simulink model "UAV_Load_Balancing_Main"  (R2025b)
settings: Solver=ode23t  StartTime=0.0  StopTime=8  FixedStep=1e-5  MaxStep=1e-5  RelTol=1e-3
libraries: nesl_utility x67, fl_lib x49, ee_lib x36
(part 1 of 2)
settings Model: Creator=cevo_  LastModifiedBy=cevo_

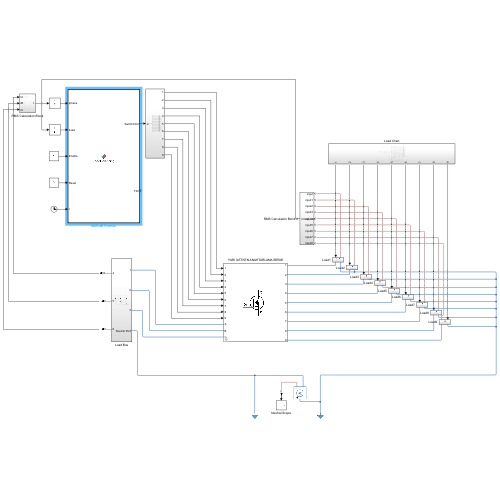
[thumbnail: Simulink's stored preview of the top-level diagram]
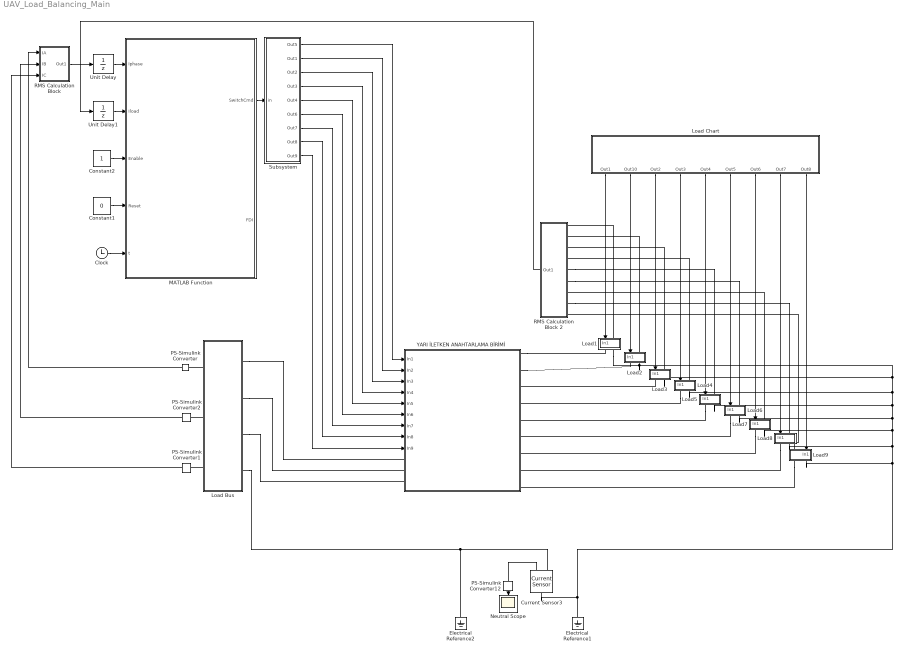
== system UAV_Load_Balancing_Main ==
  Clock : Clock
  Constant1 : Constant  Value=0
  Constant2 : Constant
  Current Sensor3 : fl_lib/Electrical/Electrical Sensors/Current Sensor
  Electrical Reference1 : fl_lib/Electrical/Electrical Elements/Electrical Reference
  Electrical Reference2 : fl_lib/Electrical/Electrical Elements/Electrical Reference
  Load Bus : Subsystem
  Load Chart : Subsystem
  Load1 : Subsystem
  Load2 : Subsystem
  Load3 : Subsystem
  Load4 : Subsystem
  Load5 : Subsystem
  Load6 : Subsystem
  Load7 : Subsystem
  Load8 : Subsystem
  Load9 : Subsystem
      settings: PortSchema="{\"entries\":[{\"content\":{\"sides\":[{\"content\":{\"connectorIds\":[\"LConn1\",\"In1\"]},\"type\":\"ConnectorPlacement.EquallySpacedRectSide\",\"uuid\":\"d3e55c95-e0b0-4c19-a363-030e817358eb\"},{\"content\":{\"connectorIds\":[\"RConn1\",\"RConn2\"],\"side\":\"RIGHT\"},\"type\":\"ConnectorPlacement.EquallySpacedRectSide\",\"uuid\":\"a0e4c3e1-714c-47ca-a01a-393fa4d5956a\"},{\"content\":{\"side\":\"TOP\"},\"type\":\"ConnectorPlacement.EquallySpacedRectSide\",\"uuid\":\"b8c3a6c7-6915-4d93-933f-da8484f2cfda\"}]},\"type\":\"ConnectorPlacement.EquallySpacedConnector\",\"uuid\":\"988140d9-c12a-4da7-b803-ba7ebfbbead4\"}],\"packageUris\":[\"http://schema.mathworks.com/mf0/Connector/R2020b\"],\"version\":\"1.0\"}"
  MATLAB Function : MATLAB Function  TreatAsAtomicUnit=on
  Neutral Scope : Scope
      settings: ActiveDisplayYMinimum=-0.021583988846100941  ActiveDisplayYMaximum=0.036156729353894947  DataLoggingVariableName=ScopeData14
  PS-Simulink Converter : nesl_utility/PS-Simulink Converter  PhysicalDomain=network_engine_domain  SubClassName=ps_output  LeftPortType=input  RightPortType=output  PseudoPeriodic=off  Frequencies=[]  VectorFormat=inherit  Unit=inherit  AffineConversion=off
  PS-Simulink Converter1 : nesl_utility/PS-Simulink Converter  PhysicalDomain=network_engine_domain  SubClassName=ps_output  LeftPortType=input  RightPortType=output  PseudoPeriodic=off  Frequencies=[]  VectorFormat=inherit  Unit=inherit  AffineConversion=off
  PS-Simulink Converter12 : nesl_utility/PS-Simulink Converter  PhysicalDomain=network_engine_domain  SubClassName=ps_output  LeftPortType=input  RightPortType=output  PseudoPeriodic=off  Frequencies=[]  VectorFormat=inherit  Unit=A  AffineConversion=off
  PS-Simulink Converter2 : nesl_utility/PS-Simulink Converter  PhysicalDomain=network_engine_domain  SubClassName=ps_output  LeftPortType=input  RightPortType=output  PseudoPeriodic=off  Frequencies=[]  VectorFormat=inherit  Unit=inherit  AffineConversion=off
  RMS Calculation Block : Subsystem
  RMS Calculation Block 2 : Subsystem
  Subsystem : Subsystem
  Unit Delay : UnitDelay  SampleTime=-1  HasFrameUpgradeWarning=on
  Unit Delay1 : UnitDelay  SampleTime=-1  HasFrameUpgradeWarning=on
  YARI İLETKEN ANAHTARLAMA BİRİMİ : Subsystem
      mask Display: image('mosfet1.png', [0,0,0,0,50,50]);
  wires:
  Load Chart/1(Out1) -> Load1/1(In1)
  Load Chart/2(Out10) -> Load2/1(In1)
  Load Chart/3(Out2) -> Load3/1(In1)
  Load Chart/4(Out3) -> Load4/1(In1)
  Load Chart/5(Out4) -> Load5/1(In1)
  Load Chart/6(Out5) -> Load6/1(In1)
  Load Chart/7(Out6) -> Load7/1(In1)
  Load Chart/8(Out7) -> Load8/1(In1)
  Load Chart/9(Out8) -> Load9/1(In1)
  Constant1/1 -> MATLAB Function/4(Reset)
  Constant2/1 -> MATLAB Function/3(Enable)
  Subsystem/1(Out5) -> YARI İLETKEN ANAHTARLAMA BİRİMİ/1(In1)
  Subsystem/2(Out1) -> YARI İLETKEN ANAHTARLAMA BİRİMİ/2(In2)
  Subsystem/3(Out2) -> YARI İLETKEN ANAHTARLAMA BİRİMİ/3(In3)
  Subsystem/4(Out3) -> YARI İLETKEN ANAHTARLAMA BİRİMİ/4(In4)
  Subsystem/5(Out4) -> YARI İLETKEN ANAHTARLAMA BİRİMİ/5(In5)
  Subsystem/9(Out9) -> YARI İLETKEN ANAHTARLAMA BİRİMİ/9(In9)
  Subsystem/8(Out8) -> YARI İLETKEN ANAHTARLAMA BİRİMİ/8(In8)
  Subsystem/7(Out7) -> YARI İLETKEN ANAHTARLAMA BİRİMİ/7(In7)
  Subsystem/6(Out6) -> YARI İLETKEN ANAHTARLAMA BİRİMİ/6(In6)
  MATLAB Function/1(SwitchCmd) -> Subsystem/1(in)
  Unit Delay/1 -> MATLAB Function/1(Iphase)
  Unit Delay1/1 -> MATLAB Function/2(Iload)
  Clock/1 -> MATLAB Function/5(t)
  PS-Simulink Converter12/1 -> Neutral Scope/1
  PS-Simulink Converter/1 -> RMS Calculation Block/1(IA)
  PS-Simulink Converter2/1 -> RMS Calculation Block/2(IB)
  PS-Simulink Converter1/1 -> RMS Calculation Block/3(IC)
  RMS Calculation Block/1(Out1) -> Unit Delay/1
  RMS Calculation Block 2/1(Out1) -> Unit Delay1/1
  connections:
  Load Bus/RConn1 -- YARI İLETKEN ANAHTARLAMA BİRİMİ/LConn1
  Load Bus/RConn2 -- YARI İLETKEN ANAHTARLAMA BİRİMİ/LConn2
  Load Bus/RConn3 -- YARI İLETKEN ANAHTARLAMA BİRİMİ/LConn3
  YARI İLETKEN ANAHTARLAMA BİRİMİ/RConn1 -- Load1/RConn1
  YARI İLETKEN ANAHTARLAMA BİRİMİ/RConn2 -- Load2/RConn1
  Load3/RConn1 -- YARI İLETKEN ANAHTARLAMA BİRİMİ/RConn3
  Load4/RConn1 -- YARI İLETKEN ANAHTARLAMA BİRİMİ/RConn4
  Load5/RConn1 -- YARI İLETKEN ANAHTARLAMA BİRİMİ/RConn5
  Load6/RConn1 -- YARI İLETKEN ANAHTARLAMA BİRİMİ/RConn6
  Load7/RConn1 -- YARI İLETKEN ANAHTARLAMA BİRİMİ/RConn7
  Load8/RConn1 -- YARI İLETKEN ANAHTARLAMA BİRİMİ/RConn8
  Load9/RConn1 -- YARI İLETKEN ANAHTARLAMA BİRİMİ/RConn9
  Load Bus/LConn1 -- PS-Simulink Converter/LConn1
  Load Bus/LConn3 -- PS-Simulink Converter1/LConn1
  Load Bus/LConn2 -- PS-Simulink Converter2/LConn1
  PS-Simulink Converter12/LConn1 -- Current Sensor3/RConn1
  Load2/RConn2 -- Electrical Reference1/LConn1 -- Current Sensor3/LConn1 -- Load9/RConn2 -- Load8/RConn2 -- Load7/RConn2 -- Load6/RConn2 -- Load5/RConn2 -- Load4/RConn2 -- Load3/RConn2 -- Load1/RConn2
  Load Bus/RConn4 -- Electrical Reference2/LConn1 -- Current Sensor3/RConn2
  Load1/LConn1 -- RMS Calculation Block 2/LConn1
  Load2/LConn1 -- RMS Calculation Block 2/LConn2
  Load3/LConn1 -- RMS Calculation Block 2/LConn3
  Load4/LConn1 -- RMS Calculation Block 2/LConn4
  RMS Calculation Block 2/LConn5 -- Load5/LConn1
  RMS Calculation Block 2/LConn6 -- Load6/LConn1
  Load7/LConn1 -- RMS Calculation Block 2/LConn7
  RMS Calculation Block 2/LConn8 -- Load8/LConn1
  Load9/LConn1 -- RMS Calculation Block 2/LConn9

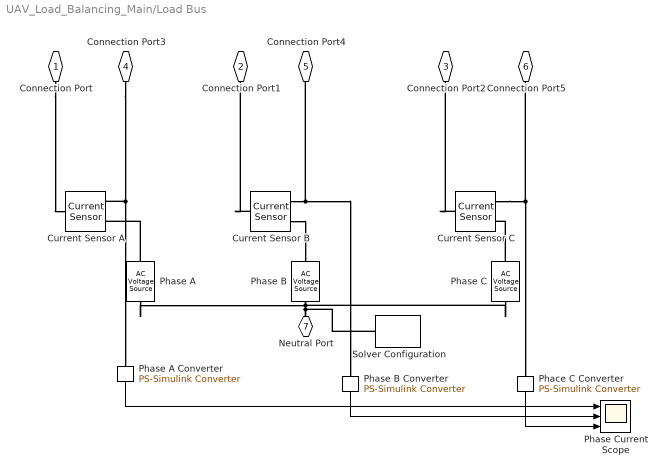
== system UAV_Load_Balancing_Main/Load Bus ==
  Current Sensor A : fl_lib/Electrical/Electrical Sensors/Current Sensor
  Current Sensor B : fl_lib/Electrical/Electrical Sensors/Current Sensor
  Current Sensor C : fl_lib/Electrical/Electrical Sensors/Current Sensor
  Phace C Converter : nesl_utility/PS-Simulink Converter  PhysicalDomain=network_engine_domain  SubClassName=ps_output  LeftPortType=input  RightPortType=output  PseudoPeriodic=off  Frequencies=[]  VectorFormat=inherit  Unit=inherit  AffineConversion=off
  Phase A : fl_lib/Electrical/Electrical Sources/AC Voltage Source  amp=115 V  shift=0 deg  frequency=400 Hz
  Phase A Converter : nesl_utility/PS-Simulink Converter  PhysicalDomain=network_engine_domain  SubClassName=ps_output  LeftPortType=input  RightPortType=output  PseudoPeriodic=off  Frequencies=[]  VectorFormat=inherit  Unit=inherit  AffineConversion=off
  Phase B : fl_lib/Electrical/Electrical Sources/AC Voltage Source  amp=115 V  shift=-120 deg  frequency=400 Hz
  Phase B Converter : nesl_utility/PS-Simulink Converter  PhysicalDomain=network_engine_domain  SubClassName=ps_output  LeftPortType=input  RightPortType=output  PseudoPeriodic=off  Frequencies=[]  VectorFormat=inherit  Unit=inherit  AffineConversion=off
  Phase C : fl_lib/Electrical/Electrical Sources/AC Voltage Source  amp=115 V  shift=120 deg  frequency=400 Hz
  Phase Current Scope : Scope  NumInputPorts=3
      settings: ActiveDisplayYMinimum=-80.91921236127051  ActiveDisplayYMaximum=82.284535528884462  DataLoggingVariableName=ScopeData16
  Solver Configuration : nesl_utility/Solver Configuration  PhysicalDomain=network_engine_domain  SubClassName=solver  LeftPortType=input  RightPortType=generic  Tones=[]  Harmonics=[]  SimulateNoise=off  Profile=off  UseLocalSampling=off  EnableSwitchedLinearOptims=on  FrequencyDomain=off  UseCCode=off  RelTol=0.001  AbsTol=0.001  MinStep=1e-09  ToWorkspace=off  RevertToSquareIcSolve=off  NumHomotopyIterations=100  PhasorMode=off  PhasorModeNumHarmonics=1  ConsistencySolver=NEWTON_XTOL_AFTER_FTOL  IndexReductionMethod=DerivativeReplacement  DoDC=off  ResidualTolerance=1e-09  ConsistencyTolSource=GLOBAL  ConsistencyAbsTol=0.001  ConsistencyRelTol=0.001  ConsistencyTolFactor=0.001  UseLocalSolver=off  LocalSolverChoice=NE_BACKWARD_EULER_ADVANCER  ResolveIndetEquations=on  FunctionEvalNumThread=1  LocalSolverSampleTime=0.001  DoFixedCost=off  MaxNonlinIter=3  MaxModeIter=2  ComputeImpulses=off  ImpulseIterations=2  LinearAlgebra=auto  LinearAlgebraNumThread=0  EquationFormulation=NE_TIME_EF  DelaysMemoryBudget=1024  AutomaticFiltering=on  FilteringTimeConstant=0.001  PartitionStorageMethod=AS_NEEDED  PartitionMemoryBudget=1024  PartitionMethod=ROBUST  MultibodyUseLocalSolver=off  MultibodyLocalSolverChoice=ODE1  MultibodyLocalSolverSampleTime=0.001
  Connection Port : PMIOPort  Side=Right
  Connection Port1 : PMIOPort  Port=2  Side=Right
  Connection Port2 : PMIOPort  Port=3  Side=Right
  Connection Port3 : PMIOPort  Port=4  Side=Left
  Connection Port4 : PMIOPort  Port=5  Side=Left
  Connection Port5 : PMIOPort  Port=6  Side=Left
  Neutral Port : PMIOPort  Port=7  Side=Right
  wires:
  Phase A Converter/1 -> Phase Current Scope/1
  Phace C Converter/1 -> Phase Current Scope/3
  Phase B Converter/1 -> Phase Current Scope/2
  connections:
  Phase C/RConn1 -- Phase B/RConn1 -- Solver Configuration/RConn1 -- Neutral Port/RConn1 -- Phase A/RConn1
  Connection Port/RConn1 -- Current Sensor A/LConn1
  Phase C/LConn1 -- Current Sensor C/RConn2
  Current Sensor B/LConn1 -- Connection Port1/RConn1
  Current Sensor C/LConn1 -- Connection Port2/RConn1
  Current Sensor B/RConn1 -- Connection Port4/RConn1 -- Phase B Converter/LConn1
  Current Sensor C/RConn1 -- Phace C Converter/LConn1 -- Connection Port5/RConn1
  Connection Port3/RConn1 -- Current Sensor A/RConn1 -- Phase A Converter/LConn1
  Phase A/LConn1 -- Current Sensor A/RConn2
  Current Sensor B/RConn2 -- Phase B/LConn1

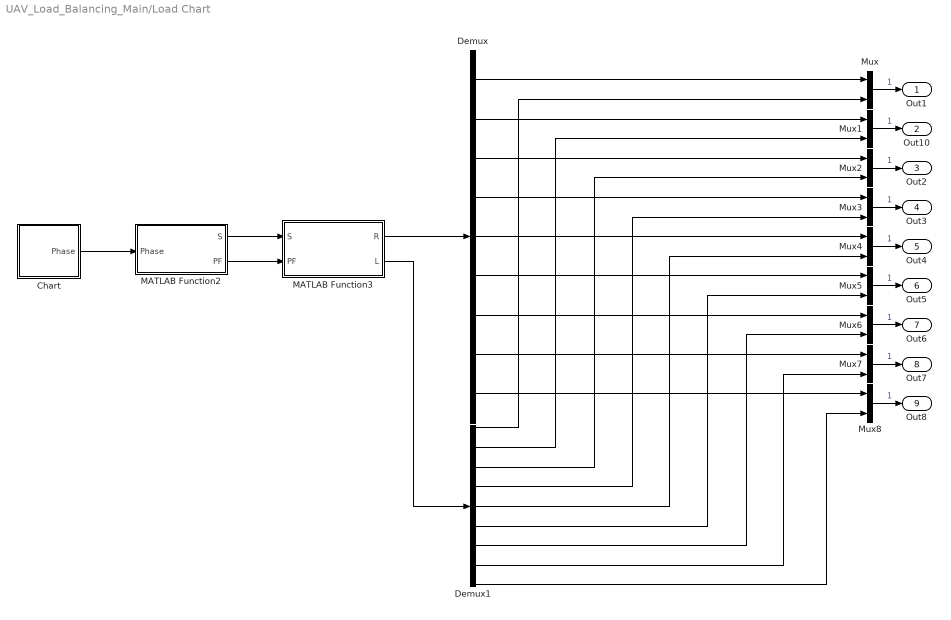
== system UAV_Load_Balancing_Main/Load Chart ==
  Chart : Stateflow chart  TreatAsAtomicUnit=on
  Demux : Demux  Outputs=9
  Demux1 : Demux  Outputs=9
  MATLAB Function2 : MATLAB Function  TreatAsAtomicUnit=on
  MATLAB Function3 : MATLAB Function  TreatAsAtomicUnit=on
  Mux{,1..8} (9 alike) : Mux  Inputs=2
  Out1 : Outport
  Out10 : Outport  Port=2
  Out2 : Outport  Port=3
  Out3 : Outport  Port=4
  Out4 : Outport  Port=5
  Out5 : Outport  Port=6
  Out6 : Outport  Port=7
  Out7 : Outport  Port=8
  Out8 : Outport  Port=9
  wires:
  Demux1/2 -> Mux1/2
  Demux1/4 -> Mux3/2
  Demux1/1 -> Mux/2
  MATLAB Function2/1(S) -> MATLAB Function3/1(S)
  MATLAB Function3/2(L) -> Demux1/1
  Demux/6 -> Mux5/1
  Chart/1(Phase) -> MATLAB Function2/1(Phase)
  Demux/2 -> Mux1/1
  MATLAB Function2/2(PF) -> MATLAB Function3/2(PF)
  MATLAB Function3/1(R) -> Demux/1
  Demux1/5 -> Mux4/2
  Demux1/3 -> Mux2/2
  Demux/1 -> Mux/1
  Demux/7 -> Mux6/1
  Demux1/8 -> Mux7/2
  Demux1/6 -> Mux5/2
  Demux1/9 -> Mux8/2
  Demux/3 -> Mux2/1
  Demux/5 -> Mux4/1
  Demux/4 -> Mux3/1
  Mux/1 -> Out1/1  "1"
  Mux1/1 -> Out10/1  "1"
  Mux2/1 -> Out2/1  "1"
  Mux3/1 -> Out3/1  "1"
  Mux4/1 -> Out4/1  "1"
  Mux6/1 -> Out6/1  "1"
  Mux7/1 -> Out7/1  "1"
  Mux5/1 -> Out5/1  "1"
  Mux8/1 -> Out8/1  "1"
  Demux/8 -> Mux7/1
  Demux/9 -> Mux8/1
  Demux1/7 -> Mux6/2

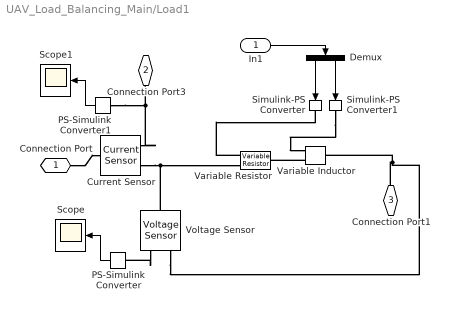
== system UAV_Load_Balancing_Main/Load1 ==
  In1 : Inport
  Current Sensor : fl_lib/Electrical/Electrical Sensors/Current Sensor
  Demux : Demux  Outputs=2
  PS-Simulink Converter : nesl_utility/PS-Simulink Converter  PhysicalDomain=network_engine_domain  SubClassName=ps_output  LeftPortType=input  RightPortType=output  PseudoPeriodic=off  Frequencies=[]  VectorFormat=inherit  Unit=inherit  AffineConversion=off
  PS-Simulink Converter1 : nesl_utility/PS-Simulink Converter  PhysicalDomain=network_engine_domain  SubClassName=ps_output  LeftPortType=input  RightPortType=output  PseudoPeriodic=off  Frequencies=[]  VectorFormat=inherit  Unit=inherit  AffineConversion=off
  Scope : Scope
      settings: ActiveDisplayYMinimum=-986.09997424371284  ActiveDisplayYMaximum=904.23363471267135
  Scope1 : Scope
      settings: ActiveDisplayYMinimum=-22.033599646280507  ActiveDisplayYMaximum=54.820487440929263
  Simulink-PS Converter : nesl_utility/Simulink-PS Converter  PhysicalDomain=network_engine_domain  SubClassName=ps_input  LeftPortType=input  RightPortType=output  PseudoPeriodic=off  Frequencies=[]  NoiseDistribution=none  NoiseParameters=[]  Unit=1  AffineConversion=off  FilteringAndDerivatives=provide  SimscapeFilterOrder=1  InputFilterTimeConstant=0.001  UdotUserProvided=0
  Simulink-PS Converter1 : nesl_utility/Simulink-PS Converter  PhysicalDomain=network_engine_domain  SubClassName=ps_input  LeftPortType=input  RightPortType=output  PseudoPeriodic=off  Frequencies=[]  NoiseDistribution=none  NoiseParameters=[]  Unit=1  AffineConversion=off  FilteringAndDerivatives=provide  SimscapeFilterOrder=1  InputFilterTimeConstant=0.001  UdotUserProvided=0
  Variable Inductor : ee_lib/Passive/Variable Inductor  prm=2  Lmin=1e-6 H  g=1e-9 1/Ohm  i0=0 A  phi0=0 Wb
      settings: InternalSimscapePortConfiguration="{\"Bottom\":[],\"Left\":[{\"id\":\"L\",\"label\":\"L\",\"type\":\"input\"},{\"id\":\"p\",\"label\":\"+\",\"type\":\"foundation.electrical.electrical\"}],\"Right\":[{\"id\":\"n\",\"label\":\"-\",\"type\":\"foundation.electrical.electrical\"}],\"Top\":[]}"
  Variable Resistor : fl_lib/Electrical/Electrical Elements/Variable Resistor  Rmin=0 Ohm  thermalEnable=false  thermal_mass=1 J/K  i_specify=off  i_priority=None  i=0 A  i_nominal_specify=off  i_nominal_value=1  i_nominal_unit=A  v_specify=off  v_priority=None  v=0 V  v_nominal_specify=off  v_nominal_value=1  v_nominal_unit=V  T_specify=off  T_priority=None  T=300 K  T_nominal_specify=off  T_nominal_value=1  T_nominal_unit=K
  Voltage Sensor : fl_lib/Electrical/Electrical Sensors/Voltage Sensor
  Connection Port : PMIOPort  Side=Right
  Connection Port3 : PMIOPort  Port=2  Side=Left
  Connection Port1 : PMIOPort  Port=3  Side=Right
  wires:
  In1/1 -> Demux/1
  PS-Simulink Converter/1 -> Scope/1
  PS-Simulink Converter1/1 -> Scope1/1
  Demux/1 -> Simulink-PS Converter/1
  Demux/2 -> Simulink-PS Converter1/1
  connections:
  Variable Resistor/LConn1 -- Simulink-PS Converter/RConn1
  Simulink-PS Converter1/RConn1 -- Variable Inductor/LConn1
  Connection Port/RConn1 -- Current Sensor/LConn1
  Voltage Sensor/RConn2 -- Connection Port1/RConn1 -- Variable Inductor/RConn1
  Current Sensor/RConn1 -- PS-Simulink Converter1/LConn1 -- Connection Port3/RConn1
  Current Sensor/RConn2 -- Variable Resistor/LConn2 -- Voltage Sensor/LConn1
  Voltage Sensor/RConn1 -- PS-Simulink Converter/LConn1
  Variable Inductor/LConn2 -- Variable Resistor/RConn1

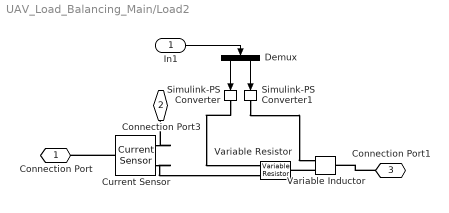
== system UAV_Load_Balancing_Main/Load2 ==
  In1 : Inport
  Current Sensor : fl_lib/Electrical/Electrical Sensors/Current Sensor
  Demux : Demux  Outputs=2
  Simulink-PS Converter : nesl_utility/Simulink-PS Converter  PhysicalDomain=network_engine_domain  SubClassName=ps_input  LeftPortType=input  RightPortType=output  PseudoPeriodic=off  Frequencies=[]  NoiseDistribution=none  NoiseParameters=[]  Unit=1  AffineConversion=off  FilteringAndDerivatives=provide  SimscapeFilterOrder=1  InputFilterTimeConstant=0.001  UdotUserProvided=0
  Simulink-PS Converter1 : nesl_utility/Simulink-PS Converter  PhysicalDomain=network_engine_domain  SubClassName=ps_input  LeftPortType=input  RightPortType=output  PseudoPeriodic=off  Frequencies=[]  NoiseDistribution=none  NoiseParameters=[]  Unit=1  AffineConversion=off  FilteringAndDerivatives=provide  SimscapeFilterOrder=1  InputFilterTimeConstant=0.001  UdotUserProvided=0
  Variable Inductor : ee_lib/Passive/Variable Inductor  prm=1  Lmin=1e-6 H  g=1e-9 1/Ohm  i0=0 A  phi0=0 Wb
      settings: InternalSimscapePortConfiguration="{\"Bottom\":[],\"Left\":[{\"id\":\"L\",\"label\":\"L\",\"type\":\"input\"},{\"id\":\"p\",\"label\":\"+\",\"type\":\"foundation.electrical.electrical\"}],\"Right\":[{\"id\":\"n\",\"label\":\"-\",\"type\":\"foundation.electrical.electrical\"}],\"Top\":[]}"
  Variable Resistor : fl_lib/Electrical/Electrical Elements/Variable Resistor  Rmin=0 Ohm  thermalEnable=false  thermal_mass=1 J/K  i_specify=off  i_priority=None  i=0 A  i_nominal_specify=off  i_nominal_value=1  i_nominal_unit=A  v_specify=off  v_priority=None  v=0 V  v_nominal_specify=off  v_nominal_value=1  v_nominal_unit=V  T_specify=off  T_priority=None  T=300 K  T_nominal_specify=off  T_nominal_value=1  T_nominal_unit=K
  Connection Port : PMIOPort  Side=Right
  Connection Port3 : PMIOPort  Port=2  Side=Left
  Connection Port1 : PMIOPort  Port=3  Side=Right
  wires:
  In1/1 -> Demux/1
  Demux/1 -> Simulink-PS Converter/1
  Demux/2 -> Simulink-PS Converter1/1
  connections:
  Simulink-PS Converter/RConn1 -- Variable Resistor/LConn1
  Simulink-PS Converter1/RConn1 -- Variable Inductor/LConn1
  Current Sensor/LConn1 -- Connection Port/RConn1
  Current Sensor/RConn1 -- Connection Port3/RConn1
  Current Sensor/RConn2 -- Variable Resistor/LConn2
  Connection Port1/RConn1 -- Variable Inductor/RConn1
  Variable Inductor/LConn2 -- Variable Resistor/RConn1

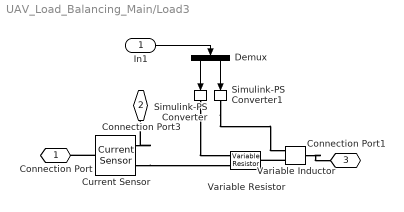
== system UAV_Load_Balancing_Main/Load3 ==
  In1 : Inport
  Current Sensor : fl_lib/Electrical/Electrical Sensors/Current Sensor
  Demux : Demux  Outputs=2
  Simulink-PS Converter : nesl_utility/Simulink-PS Converter  PhysicalDomain=network_engine_domain  SubClassName=ps_input  LeftPortType=input  RightPortType=output  PseudoPeriodic=off  Frequencies=[]  NoiseDistribution=none  NoiseParameters=[]  Unit=1  AffineConversion=off  FilteringAndDerivatives=provide  SimscapeFilterOrder=1  InputFilterTimeConstant=0.001  UdotUserProvided=0
  Simulink-PS Converter1 : nesl_utility/Simulink-PS Converter  PhysicalDomain=network_engine_domain  SubClassName=ps_input  LeftPortType=input  RightPortType=output  PseudoPeriodic=off  Frequencies=[]  NoiseDistribution=none  NoiseParameters=[]  Unit=1  AffineConversion=off  FilteringAndDerivatives=provide  SimscapeFilterOrder=1  InputFilterTimeConstant=0.001  UdotUserProvided=0
  Variable Inductor : ee_lib/Passive/Variable Inductor  prm=1  Lmin=1e-6 H  g=1e-9 1/Ohm  i0=0 A  phi0=0 Wb
      settings: InternalSimscapePortConfiguration="{\"Bottom\":[],\"Left\":[{\"id\":\"L\",\"label\":\"L\",\"type\":\"input\"},{\"id\":\"p\",\"label\":\"+\",\"type\":\"foundation.electrical.electrical\"}],\"Right\":[{\"id\":\"n\",\"label\":\"-\",\"type\":\"foundation.electrical.electrical\"}],\"Top\":[]}"
  Variable Resistor : fl_lib/Electrical/Electrical Elements/Variable Resistor  Rmin=0 Ohm  thermalEnable=false  thermal_mass=1 J/K  i_specify=off  i_priority=None  i=0 A  i_nominal_specify=off  i_nominal_value=1  i_nominal_unit=A  v_specify=off  v_priority=None  v=0 V  v_nominal_specify=off  v_nominal_value=1  v_nominal_unit=V  T_specify=off  T_priority=None  T=300 K  T_nominal_specify=off  T_nominal_value=1  T_nominal_unit=K
  Connection Port : PMIOPort  Side=Right
  Connection Port3 : PMIOPort  Port=2  Side=Left
  Connection Port1 : PMIOPort  Port=3  Side=Right
  wires:
  In1/1 -> Demux/1
  Demux/1 -> Simulink-PS Converter/1
  Demux/2 -> Simulink-PS Converter1/1
  connections:
  Simulink-PS Converter/RConn1 -- Variable Resistor/LConn1
  Simulink-PS Converter1/RConn1 -- Variable Inductor/LConn1
  Current Sensor/LConn1 -- Connection Port/RConn1
  Current Sensor/RConn1 -- Connection Port3/RConn1
  Current Sensor/RConn2 -- Variable Resistor/LConn2
  Variable Inductor/LConn2 -- Variable Resistor/RConn1
  Variable Inductor/RConn1 -- Connection Port1/RConn1

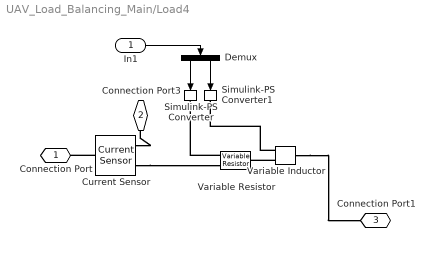
== system UAV_Load_Balancing_Main/Load4 ==
  In1 : Inport
  Current Sensor : fl_lib/Electrical/Electrical Sensors/Current Sensor
  Demux : Demux  Outputs=2
  Simulink-PS Converter : nesl_utility/Simulink-PS Converter  PhysicalDomain=network_engine_domain  SubClassName=ps_input  LeftPortType=input  RightPortType=output  PseudoPeriodic=off  Frequencies=[]  NoiseDistribution=none  NoiseParameters=[]  Unit=1  AffineConversion=off  FilteringAndDerivatives=provide  SimscapeFilterOrder=1  InputFilterTimeConstant=0.001  UdotUserProvided=0
  Simulink-PS Converter1 : nesl_utility/Simulink-PS Converter  PhysicalDomain=network_engine_domain  SubClassName=ps_input  LeftPortType=input  RightPortType=output  PseudoPeriodic=off  Frequencies=[]  NoiseDistribution=none  NoiseParameters=[]  Unit=1  AffineConversion=off  FilteringAndDerivatives=provide  SimscapeFilterOrder=1  InputFilterTimeConstant=0.001  UdotUserProvided=0
  Variable Inductor : ee_lib/Passive/Variable Inductor  prm=1  Lmin=1e-6 H  g=1e-9 1/Ohm  i0=0 A  phi0=0 Wb
      settings: InternalSimscapePortConfiguration="{\"Bottom\":[],\"Left\":[{\"id\":\"L\",\"label\":\"L\",\"type\":\"input\"},{\"id\":\"p\",\"label\":\"+\",\"type\":\"foundation.electrical.electrical\"}],\"Right\":[{\"id\":\"n\",\"label\":\"-\",\"type\":\"foundation.electrical.electrical\"}],\"Top\":[]}"
  Variable Resistor : fl_lib/Electrical/Electrical Elements/Variable Resistor  Rmin=0 Ohm  thermalEnable=false  thermal_mass=1 J/K  i_specify=off  i_priority=None  i=0 A  i_nominal_specify=off  i_nominal_value=1  i_nominal_unit=A  v_specify=off  v_priority=None  v=0 V  v_nominal_specify=off  v_nominal_value=1  v_nominal_unit=V  T_specify=off  T_priority=None  T=300 K  T_nominal_specify=off  T_nominal_value=1  T_nominal_unit=K
  Connection Port : PMIOPort  Side=Right
  Connection Port3 : PMIOPort  Port=2  Side=Left
  Connection Port1 : PMIOPort  Port=3  Side=Right
  wires:
  In1/1 -> Demux/1
  Demux/1 -> Simulink-PS Converter/1
  Demux/2 -> Simulink-PS Converter1/1
  connections:
  Current Sensor/LConn1 -- Connection Port/RConn1
  Current Sensor/RConn1 -- Connection Port3/RConn1
  Current Sensor/RConn2 -- Variable Resistor/LConn2
  Variable Inductor/LConn1 -- Simulink-PS Converter1/RConn1
  Variable Resistor/LConn1 -- Simulink-PS Converter/RConn1
  Variable Inductor/LConn2 -- Variable Resistor/RConn1
  Variable Inductor/RConn1 -- Connection Port1/RConn1

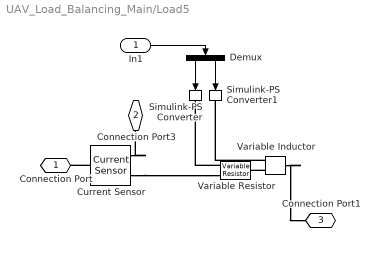
== system UAV_Load_Balancing_Main/Load5 ==
  In1 : Inport
  Current Sensor : fl_lib/Electrical/Electrical Sensors/Current Sensor
  Demux : Demux  Outputs=2
  Simulink-PS Converter : nesl_utility/Simulink-PS Converter  PhysicalDomain=network_engine_domain  SubClassName=ps_input  LeftPortType=input  RightPortType=output  PseudoPeriodic=off  Frequencies=[]  NoiseDistribution=none  NoiseParameters=[]  Unit=1  AffineConversion=off  FilteringAndDerivatives=provide  SimscapeFilterOrder=1  InputFilterTimeConstant=0.001  UdotUserProvided=0
  Simulink-PS Converter1 : nesl_utility/Simulink-PS Converter  PhysicalDomain=network_engine_domain  SubClassName=ps_input  LeftPortType=input  RightPortType=output  PseudoPeriodic=off  Frequencies=[]  NoiseDistribution=none  NoiseParameters=[]  Unit=1  AffineConversion=off  FilteringAndDerivatives=provide  SimscapeFilterOrder=1  InputFilterTimeConstant=0.001  UdotUserProvided=0
  Variable Inductor : ee_lib/Passive/Variable Inductor  prm=1  Lmin=1e-6 H  g=1e-9 1/Ohm  i0=0 A  phi0=0 Wb
      settings: InternalSimscapePortConfiguration="{\"Bottom\":[],\"Left\":[{\"id\":\"L\",\"label\":\"L\",\"type\":\"input\"},{\"id\":\"p\",\"label\":\"+\",\"type\":\"foundation.electrical.electrical\"}],\"Right\":[{\"id\":\"n\",\"label\":\"-\",\"type\":\"foundation.electrical.electrical\"}],\"Top\":[]}"
  Variable Resistor : fl_lib/Electrical/Electrical Elements/Variable Resistor  Rmin=0 Ohm  thermalEnable=false  thermal_mass=1 J/K  i_specify=off  i_priority=None  i=0 A  i_nominal_specify=off  i_nominal_value=1  i_nominal_unit=A  v_specify=off  v_priority=None  v=0 V  v_nominal_specify=off  v_nominal_value=1  v_nominal_unit=V  T_specify=off  T_priority=None  T=300 K  T_nominal_specify=off  T_nominal_value=1  T_nominal_unit=K
  Connection Port : PMIOPort  Side=Right
  Connection Port3 : PMIOPort  Port=2  Side=Left
  Connection Port1 : PMIOPort  Port=3  Side=Right
  wires:
  In1/1 -> Demux/1
  Demux/1 -> Simulink-PS Converter/1
  Demux/2 -> Simulink-PS Converter1/1
  connections:
  Current Sensor/LConn1 -- Connection Port/RConn1
  Current Sensor/RConn1 -- Connection Port3/RConn1
  Current Sensor/RConn2 -- Variable Resistor/LConn2
  Variable Inductor/LConn1 -- Simulink-PS Converter1/RConn1
  Variable Resistor/LConn1 -- Simulink-PS Converter/RConn1
  Variable Inductor/LConn2 -- Variable Resistor/RConn1
  Variable Inductor/RConn1 -- Connection Port1/RConn1

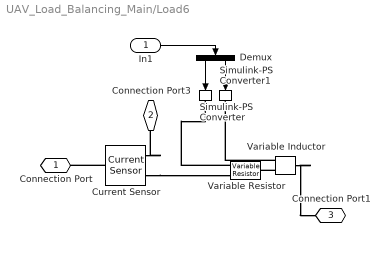
== system UAV_Load_Balancing_Main/Load6 ==
  In1 : Inport
  Current Sensor : fl_lib/Electrical/Electrical Sensors/Current Sensor
  Demux : Demux  Outputs=2
  Simulink-PS Converter : nesl_utility/Simulink-PS Converter  PhysicalDomain=network_engine_domain  SubClassName=ps_input  LeftPortType=input  RightPortType=output  PseudoPeriodic=off  Frequencies=[]  NoiseDistribution=none  NoiseParameters=[]  Unit=1  AffineConversion=off  FilteringAndDerivatives=provide  SimscapeFilterOrder=1  InputFilterTimeConstant=0.001  UdotUserProvided=0
  Simulink-PS Converter1 : nesl_utility/Simulink-PS Converter  PhysicalDomain=network_engine_domain  SubClassName=ps_input  LeftPortType=input  RightPortType=output  PseudoPeriodic=off  Frequencies=[]  NoiseDistribution=none  NoiseParameters=[]  Unit=1  AffineConversion=off  FilteringAndDerivatives=provide  SimscapeFilterOrder=1  InputFilterTimeConstant=0.001  UdotUserProvided=0
  Variable Inductor : ee_lib/Passive/Variable Inductor  prm=1  Lmin=1e-6 H  g=1e-9 1/Ohm  i0=0 A  phi0=0 Wb
      settings: InternalSimscapePortConfiguration="{\"Bottom\":[],\"Left\":[{\"id\":\"L\",\"label\":\"L\",\"type\":\"input\"},{\"id\":\"p\",\"label\":\"+\",\"type\":\"foundation.electrical.electrical\"}],\"Right\":[{\"id\":\"n\",\"label\":\"-\",\"type\":\"foundation.electrical.electrical\"}],\"Top\":[]}"
  Variable Resistor : fl_lib/Electrical/Electrical Elements/Variable Resistor  Rmin=0 Ohm  thermalEnable=false  thermal_mass=1 J/K  i_specify=off  i_priority=None  i=0 A  i_nominal_specify=off  i_nominal_value=1  i_nominal_unit=A  v_specify=off  v_priority=None  v=0 V  v_nominal_specify=off  v_nominal_value=1  v_nominal_unit=V  T_specify=off  T_priority=None  T=300 K  T_nominal_specify=off  T_nominal_value=1  T_nominal_unit=K
  Connection Port : PMIOPort  Side=Right
  Connection Port3 : PMIOPort  Port=2  Side=Left
  Connection Port1 : PMIOPort  Port=3  Side=Right
  wires:
  In1/1 -> Demux/1
  Demux/1 -> Simulink-PS Converter/1
  Demux/2 -> Simulink-PS Converter1/1
  connections:
  Current Sensor/LConn1 -- Connection Port/RConn1
  Current Sensor/RConn1 -- Connection Port3/RConn1
  Current Sensor/RConn2 -- Variable Resistor/LConn2
  Variable Inductor/LConn1 -- Simulink-PS Converter1/RConn1
  Variable Resistor/LConn1 -- Simulink-PS Converter/RConn1
  Variable Inductor/LConn2 -- Variable Resistor/RConn1
  Variable Inductor/RConn1 -- Connection Port1/RConn1

== system UAV_Load_Balancing_Main/Load7 ==
  In1 : Inport
  Current Sensor : fl_lib/Electrical/Electrical Sensors/Current Sensor
  Demux : Demux  Outputs=2
  Simulink-PS Converter : nesl_utility/Simulink-PS Converter  PhysicalDomain=network_engine_domain  SubClassName=ps_input  LeftPortType=input  RightPortType=output  PseudoPeriodic=off  Frequencies=[]  NoiseDistribution=none  NoiseParameters=[]  Unit=1  AffineConversion=off  FilteringAndDerivatives=provide  SimscapeFilterOrder=1  InputFilterTimeConstant=0.001  UdotUserProvided=0
  Simulink-PS Converter1 : nesl_utility/Simulink-PS Converter  PhysicalDomain=network_engine_domain  SubClassName=ps_input  LeftPortType=input  RightPortType=output  PseudoPeriodic=off  Frequencies=[]  NoiseDistribution=none  NoiseParameters=[]  Unit=1  AffineConversion=off  FilteringAndDerivatives=provide  SimscapeFilterOrder=1  InputFilterTimeConstant=0.001  UdotUserProvided=0
  Variable Inductor : ee_lib/Passive/Variable Inductor  prm=1  Lmin=1e-6 H  g=1e-9 1/Ohm  i0=0 A  phi0=0 Wb
      settings: InternalSimscapePortConfiguration="{\"Bottom\":[],\"Left\":[{\"id\":\"L\",\"label\":\"L\",\"type\":\"input\"},{\"id\":\"p\",\"label\":\"+\",\"type\":\"foundation.electrical.electrical\"}],\"Right\":[{\"id\":\"n\",\"label\":\"-\",\"type\":\"foundation.electrical.electrical\"}],\"Top\":[]}"
  Variable Resistor : fl_lib/Electrical/Electrical Elements/Variable Resistor  Rmin=0 Ohm  thermalEnable=false  thermal_mass=1 J/K  i_specify=off  i_priority=None  i=0 A  i_nominal_specify=off  i_nominal_value=1  i_nominal_unit=A  v_specify=off  v_priority=None  v=0 V  v_nominal_specify=off  v_nominal_value=1  v_nominal_unit=V  T_specify=off  T_priority=None  T=300 K  T_nominal_specify=off  T_nominal_value=1  T_nominal_unit=K
  Connection Port : PMIOPort  Side=Right
  Connection Port3 : PMIOPort  Port=2  Side=Left
  Connection Port1 : PMIOPort  Port=3  Side=Right
  wires:
  In1/1 -> Demux/1
  Demux/1 -> Simulink-PS Converter/1
  Demux/2 -> Simulink-PS Converter1/1
  connections:
  Current Sensor/LConn1 -- Connection Port/RConn1
  Current Sensor/RConn1 -- Connection Port3/RConn1
  Current Sensor/RConn2 -- Variable Resistor/LConn2
  Simulink-PS Converter1/RConn1 -- Variable Inductor/LConn1
  Simulink-PS Converter/RConn1 -- Variable Resistor/LConn1
  Variable Inductor/LConn2 -- Variable Resistor/RConn1
  Variable Inductor/RConn1 -- Connection Port1/RConn1

== system UAV_Load_Balancing_Main/Load8 ==
  In1 : Inport
  Current Sensor : fl_lib/Electrical/Electrical Sensors/Current Sensor
  Demux : Demux  Outputs=2
  Simulink-PS Converter : nesl_utility/Simulink-PS Converter  PhysicalDomain=network_engine_domain  SubClassName=ps_input  LeftPortType=input  RightPortType=output  PseudoPeriodic=off  Frequencies=[]  NoiseDistribution=none  NoiseParameters=[]  Unit=1  AffineConversion=off  FilteringAndDerivatives=provide  SimscapeFilterOrder=1  InputFilterTimeConstant=0.001  UdotUserProvided=0
  Simulink-PS Converter1 : nesl_utility/Simulink-PS Converter  PhysicalDomain=network_engine_domain  SubClassName=ps_input  LeftPortType=input  RightPortType=output  PseudoPeriodic=off  Frequencies=[]  NoiseDistribution=none  NoiseParameters=[]  Unit=1  AffineConversion=off  FilteringAndDerivatives=provide  SimscapeFilterOrder=1  InputFilterTimeConstant=0.001  UdotUserProvided=0
  Variable Inductor : ee_lib/Passive/Variable Inductor  prm=1  Lmin=1e-6 H  g=1e-9 1/Ohm  i0=0 A  phi0=0 Wb
      settings: InternalSimscapePortConfiguration="{\"Bottom\":[],\"Left\":[{\"id\":\"L\",\"label\":\"L\",\"type\":\"input\"},{\"id\":\"p\",\"label\":\"+\",\"type\":\"foundation.electrical.electrical\"}],\"Right\":[{\"id\":\"n\",\"label\":\"-\",\"type\":\"foundation.electrical.electrical\"}],\"Top\":[]}"
  Variable Resistor : fl_lib/Electrical/Electrical Elements/Variable Resistor  Rmin=0 Ohm  thermalEnable=false  thermal_mass=1 J/K  i_specify=off  i_priority=None  i=0 A  i_nominal_specify=off  i_nominal_value=1  i_nominal_unit=A  v_specify=off  v_priority=None  v=0 V  v_nominal_specify=off  v_nominal_value=1  v_nominal_unit=V  T_specify=off  T_priority=None  T=300 K  T_nominal_specify=off  T_nominal_value=1  T_nominal_unit=K
  Connection Port : PMIOPort  Side=Right
  Connection Port3 : PMIOPort  Port=2  Side=Left
  Connection Port1 : PMIOPort  Port=3  Side=Right
  wires:
  In1/1 -> Demux/1
  Demux/1 -> Simulink-PS Converter/1
  Demux/2 -> Simulink-PS Converter1/1
  connections:
  Current Sensor/LConn1 -- Connection Port/RConn1
  Current Sensor/RConn1 -- Connection Port3/RConn1
  Current Sensor/RConn2 -- Variable Resistor/LConn2
  Variable Inductor/LConn1 -- Simulink-PS Converter1/RConn1
  Variable Resistor/LConn1 -- Simulink-PS Converter/RConn1
  Variable Inductor/LConn2 -- Variable Resistor/RConn1
  Connection Port1/RConn1 -- Variable Inductor/RConn1

== system UAV_Load_Balancing_Main/Load9 ==
  In1 : Inport
  Current Sensor : fl_lib/Electrical/Electrical Sensors/Current Sensor
  Demux : Demux  Outputs=2
  Simulink-PS Converter : nesl_utility/Simulink-PS Converter  PhysicalDomain=network_engine_domain  SubClassName=ps_input  LeftPortType=input  RightPortType=output  PseudoPeriodic=off  Frequencies=[]  NoiseDistribution=none  NoiseParameters=[]  Unit=1  AffineConversion=off  FilteringAndDerivatives=provide  SimscapeFilterOrder=1  InputFilterTimeConstant=0.001  UdotUserProvided=0
  Simulink-PS Converter1 : nesl_utility/Simulink-PS Converter  PhysicalDomain=network_engine_domain  SubClassName=ps_input  LeftPortType=input  RightPortType=output  PseudoPeriodic=off  Frequencies=[]  NoiseDistribution=none  NoiseParameters=[]  Unit=1  AffineConversion=off  FilteringAndDerivatives=provide  SimscapeFilterOrder=1  InputFilterTimeConstant=0.001  UdotUserProvided=0
  Variable Inductor : ee_lib/Passive/Variable Inductor  prm=1  Lmin=1e-6 H  g=1e-9 1/Ohm  i0=0 A  phi0=0 Wb
      settings: InternalSimscapePortConfiguration="{\"Bottom\":[],\"Left\":[{\"id\":\"L\",\"label\":\"L\",\"type\":\"input\"},{\"id\":\"p\",\"label\":\"+\",\"type\":\"foundation.electrical.electrical\"}],\"Right\":[{\"id\":\"n\",\"label\":\"-\",\"type\":\"foundation.electrical.electrical\"}],\"Top\":[]}"
  Variable Resistor : fl_lib/Electrical/Electrical Elements/Variable Resistor  Rmin=0 Ohm  thermalEnable=false  thermal_mass=1 J/K  i_specify=off  i_priority=None  i=0 A  i_nominal_specify=off  i_nominal_value=1  i_nominal_unit=A  v_specify=off  v_priority=None  v=0 V  v_nominal_specify=off  v_nominal_value=1  v_nominal_unit=V  T_specify=off  T_priority=None  T=300 K  T_nominal_specify=off  T_nominal_value=1  T_nominal_unit=K
  Connection Port3 : PMIOPort  Side=Left
  Connection Port1 : PMIOPort  Port=2  Side=Right
  Connection Port : PMIOPort  Port=3  Side=Right
  wires:
  In1/1 -> Demux/1
  Demux/1 -> Simulink-PS Converter/1
  Demux/2 -> Simulink-PS Converter1/1
  connections:
  Current Sensor/LConn1 -- Connection Port/RConn1
  Current Sensor/RConn1 -- Connection Port3/RConn1
  Current Sensor/RConn2 -- Variable Resistor/LConn2
  Variable Inductor/LConn1 -- Simulink-PS Converter1/RConn1
  Variable Resistor/LConn1 -- Simulink-PS Converter/RConn1
  Variable Inductor/LConn2 -- Variable Resistor/RConn1
  Variable Inductor/RConn1 -- Connection Port1/RConn1

== system UAV_Load_Balancing_Main/RMS Calculation Block ==
  IA : Inport
  IB : Inport  Port=2
  IC : Inport  Port=3
  MATLAB Function : MATLAB Function  TreatAsAtomicUnit=on
  MATLAB Function1 : MATLAB Function  TreatAsAtomicUnit=on  SystemSampleTime=1e-5
  Mux : Mux  Inputs=3
  RMS Phase Current : Scope
      settings: ActiveDisplayYMinimum=-66.770677567611727  ActiveDisplayYMaximum=393.93092204333686  DataLoggingVariableName=ScopeData2
  RMS Phase Current1 : Scope
      settings: ActiveDisplayYMinimum=2.3767747596663362  ActiveDisplayYMaximum=32.899434847118165  DataLoggingVariableName=ScopeData5
  Out1 : Outport
  wires:
  IC/1 -> MATLAB Function1/3(IC)
  MATLAB Function1/2(IrmsB) -> Mux/2
  MATLAB Function1/1(IrmsA) -> Mux/1
  MATLAB Function1/3(IrmsC) -> Mux/3
  Mux/1 -> MATLAB Function/1(Iphase), Out1/1, RMS Phase Current/1
  IB/1 -> MATLAB Function1/2(IB)
  IA/1 -> MATLAB Function1/1(IA)
  MATLAB Function/1(FDI) -> RMS Phase Current1/1

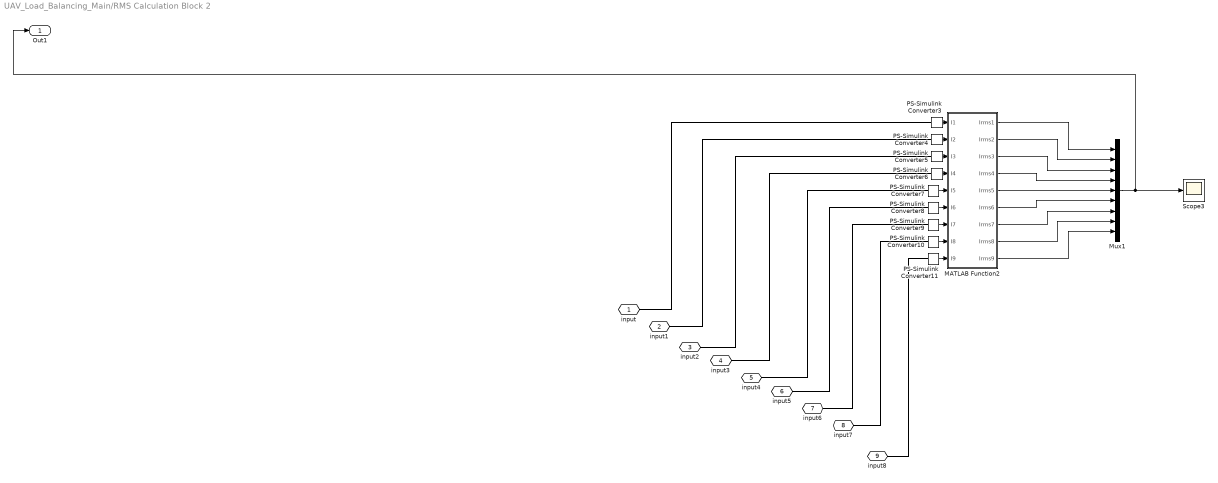
== system UAV_Load_Balancing_Main/RMS Calculation Block 2 ==
  MATLAB Function2 : MATLAB Function  TreatAsAtomicUnit=on
  Mux1 : Mux  Inputs=9
  PS-Simulink Converter{3..11} (9 alike) : nesl_utility/PS-Simulink Converter  PhysicalDomain=network_engine_domain  SubClassName=ps_output  LeftPortType=input  RightPortType=output  PseudoPeriodic=off  Frequencies=[]  VectorFormat=inherit  Unit=inherit  AffineConversion=off
  Scope3 : Scope
      settings: ActiveDisplayYMinimum=-43.363049041504865  ActiveDisplayYMaximum=311.38418436393772  DataLoggingVariableName=ScopeData3
  input : PMIOPort  Side=Left
  input1 : PMIOPort  Port=2  Side=Left
  input2 : PMIOPort  Port=3  Side=Left
  input3 : PMIOPort  Port=4  Side=Left
  input4 : PMIOPort  Port=5  Side=Left
  input5 : PMIOPort  Port=6  Side=Left
  input6 : PMIOPort  Port=7  Side=Left
  input7 : PMIOPort  Port=8  Side=Left
  input8 : PMIOPort  Port=9  Side=Left
  Out1 : Outport
  wires:
  MATLAB Function2/4(Irms4) -> Mux1/4
  MATLAB Function2/9(Irms9) -> Mux1/9
  PS-Simulink Converter11/1 -> MATLAB Function2/9(I9)
  Mux1/1 -> Out1/1, Scope3/1
  PS-Simulink Converter9/1 -> MATLAB Function2/7(I7)
  MATLAB Function2/7(Irms7) -> Mux1/7
  MATLAB Function2/2(Irms2) -> Mux1/2
  MATLAB Function2/6(Irms6) -> Mux1/6
  PS-Simulink Converter6/1 -> MATLAB Function2/4(I4)
  PS-Simulink Converter3/1 -> MATLAB Function2/1(I1)
  MATLAB Function2/5(Irms5) -> Mux1/5
  PS-Simulink Converter4/1 -> MATLAB Function2/2(I2)
  PS-Simulink Converter8/1 -> MATLAB Function2/6(I6)
  MATLAB Function2/8(Irms8) -> Mux1/8
  PS-Simulink Converter5/1 -> MATLAB Function2/3(I3)
  MATLAB Function2/1(Irms1) -> Mux1/1
  PS-Simulink Converter10/1 -> MATLAB Function2/8(I8)
  MATLAB Function2/3(Irms3) -> Mux1/3
  PS-Simulink Converter7/1 -> MATLAB Function2/5(I5)
  connections:
  input/RConn1 -- PS-Simulink Converter3/LConn1
  PS-Simulink Converter8/LConn1 -- input5/RConn1
  input8/RConn1 -- PS-Simulink Converter11/LConn1
  input6/RConn1 -- PS-Simulink Converter9/LConn1
  PS-Simulink Converter7/LConn1 -- input4/RConn1
  PS-Simulink Converter10/LConn1 -- input7/RConn1
  input1/RConn1 -- PS-Simulink Converter4/LConn1
  input2/RConn1 -- PS-Simulink Converter5/LConn1
  input3/RConn1 -- PS-Simulink Converter6/LConn1

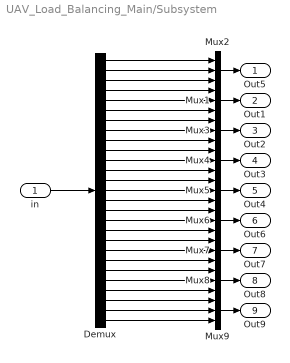
== system UAV_Load_Balancing_Main/Subsystem ==
  in : Inport
  Demux : Demux  Outputs=27
  Mux{1..9} (9 alike) : Mux  Inputs=3
  Out5 : Outport
  Out1 : Outport  Port=2
  Out2 : Outport  Port=3
  Out3 : Outport  Port=4
  Out4 : Outport  Port=5
  Out6 : Outport  Port=6
  Out7 : Outport  Port=7
  Out8 : Outport  Port=8
  Out9 : Outport  Port=9
  wires:
  Demux/5 -> Mux1/2
  Demux/25 -> Mux9/1
  Demux/26 -> Mux9/2
  Demux/21 -> Mux7/3
  Demux/18 -> Mux6/3
  Demux/20 -> Mux7/2
  Demux/23 -> Mux8/2
  Demux/22 -> Mux8/1
  Demux/3 -> Mux2/3
  Demux/24 -> Mux8/3
  Demux/9 -> Mux3/3
  in/1 -> Demux/1
  Demux/27 -> Mux9/3
  Mux2/1 -> Out5/1
  Demux/11 -> Mux4/2
  Demux/16 -> Mux6/1
  Demux/19 -> Mux7/1
  Demux/7 -> Mux3/1
  Demux/2 -> Mux2/2
  Demux/1 -> Mux2/1
  Demux/4 -> Mux1/1
  Demux/6 -> Mux1/3
  Demux/15 -> Mux5/3
  Demux/17 -> Mux6/2
  Demux/8 -> Mux3/2
  Demux/12 -> Mux4/3
  Demux/13 -> Mux5/1
  Demux/14 -> Mux5/2
  Demux/10 -> Mux4/1
  Mux1/1 -> Out1/1
  Mux3/1 -> Out2/1
  Mux4/1 -> Out3/1
  Mux5/1 -> Out4/1
  Mux6/1 -> Out6/1
  Mux7/1 -> Out7/1
  Mux8/1 -> Out8/1
  Mux9/1 -> Out9/1
